simulink model "ASM_Traffic_A11"  (R2026a)
settings: Solver=ode1  StartTime=SIM.tstart.v  StopTime=SIM.tend.v  FixedStep=SIM.StepSize.v
PostLoadFcn:
  | if any(exist('dsrtsu_mdlpostloadfcn', 'file') ~= 0), dsrtsu_mdlpostloadfcn('Execute', bdroot); end
  | try, asm_mdl_postloadfcn(bdroot, 'UpdateModel', 3600); catch, disp(lasterr); end,
InitFcn:
  | , if any(exist('rtifpga_mdlclblib', 'file') ~= 0), rtifpga_mdlclblib('Init', bdroot); end,
  | , if any(exist('dsmpb_private', 'file') ~= 0), dsmpb_private('dsmpb_mdlclblib', 'Init', bdroot); end,
undefined symbols (not defined in the file): _to_, a0b2, ASM_BrakeHydraulics_DemoSystems, ASM_VehicleDynamics_DemoSystems, b98103fe8ad365046cd0, BrakeCircuit, controllerConfig, CPT, Crankshaft, DiscIntNeverNeededParam, dsmsi, FinalDriveAssembly, instance, MDL, ModeSignals, mu, Pos_BrakePedal_Maneuver, rad, RefSignals, s_to_rpm, SIM, SoftECU, Suspension, Tire, Transmission
libraries: ASM_Traffic_lib x135, simulink x98, ASM_Utils_lib x77, ASM_VehicleDynamics_lib x70, ASM_Environment_lib x22, dsmpblib x20, dsmsilib x15, MDLD_Utils_lib x10, ASM_BrakeHydraulics_lib x3, sl_discontinuities x2
(part 43 of 63)

== system ASM_Traffic_A11/VehicleDynamics/Plant/UserInterface/DISP_Plant/Velocities ==
  Velocities : Inport
  Angle_SideSlip_Vehicle[deg] : Subsystem
      mask Display: disp('')
  AngularVelocities : Scope  NumInputPorts=3
      settings: TimeSpan=5  ActiveDisplayYMinimum=43.2  ActiveDisplayYMaximum=45.1  DataLoggingMaxPoints=20000  DataLoggingDecimation=10  DataLoggingVariableName=ScopeData67
  Bus Selector2 : BusSelector  OutputSignals=Vehicle.Linear.v_Vehicle_CoG[x;y;z][km|h].v_x_Vehicle_CoG[km|h],Vehicle.Linear.v_Vehicle_CoG[x;y;z][km|h].v_y_Vehicle_CoG[km|h],Vehicle.Linear.v_Vehicle_CoG[x;y;z][km|h].v_z_Vehicle_CoG[km|h],Vehicle.Linear.Angle_SideSlip_Vehicle[deg],Vehicle.Angular.w_Vehicle_CoG[x;y;z][deg|s].RollRate_Vehicle_CoG[deg|s],Vehicle.Angular.w_Vehicle_CoG[x;y;z][deg|s].PitchRate_Vehicle_CoG[deg|s],Vehicle.Angular.w_Vehicle_CoG[x;y;z][deg|s].YawRate_Vehicle_CoG[deg|s]
  PitchRate_Vehicle_CoG[deg|s] : Subsystem
      mask Display: disp('')
  RollRate_Vehicle_CoG[deg|s] : Subsystem
      mask Display: disp('')
  TransVelocities : Scope  NumInputPorts=4
      settings: TimeSpan=5  ActiveDisplayYMinimum=-7.51344  ActiveDisplayYMaximum=67.07764  DataLoggingMaxPoints=20000  DataLoggingDecimation=10
  YawRate_Vehicle_CoG[deg|s] : Subsystem
      mask Display: disp('')
  v_x_Vehicle_CoG[km|h] : Subsystem
      mask Display: disp('')
  v_y_Vehicle_CoG[km|h] : Subsystem
      mask Display: disp('')
  v_z_Vehicle_CoG[km|h] : Subsystem
      mask Display: disp('')
  wires:
  Velocities/1 -> Bus Selector2/1
  RollRate_Vehicle_CoG[deg|s]/1(Out1) -> AngularVelocities/1  "RollRate_Vehicle_CoG[deg|s]"
  PitchRate_Vehicle_CoG[deg|s]/1(Out1) -> AngularVelocities/2  "PitchRate_Vehicle_CoG[deg|s]"
  YawRate_Vehicle_CoG[deg|s]/1(Out1) -> AngularVelocities/3  "YawRate_Vehicle_CoG[deg|s]"
  v_x_Vehicle_CoG[km|h]/1(Out1) -> TransVelocities/1  "v_x_Vehicle_CoG[km|h]"
  v_y_Vehicle_CoG[km|h]/1(Out1) -> TransVelocities/2  "v_y_Vehicle_CoG[km|h]"
  v_z_Vehicle_CoG[km|h]/1(Out1) -> TransVelocities/3  "v_z_Vehicle_CoG[km|h]"
  Angle_SideSlip_Vehicle[deg]/1(Out1) -> TransVelocities/4  "Angle_SideSlip_Vehicle[deg]"
  Bus Selector2/1 -> v_x_Vehicle_CoG[km|h]/1(In1)  "<v_x_Vehicle_CoG[km|h]>"
  Bus Selector2/2 -> v_y_Vehicle_CoG[km|h]/1(In1)  "<v_y_Vehicle_CoG[km|h]>"
  Bus Selector2/3 -> v_z_Vehicle_CoG[km|h]/1(In1)  "<v_z_Vehicle_CoG[km|h]>"
  Bus Selector2/4 -> Angle_SideSlip_Vehicle[deg]/1(In1)  "<Angle_SideSlip_Vehicle[deg]>"
  Bus Selector2/5 -> RollRate_Vehicle_CoG[deg|s]/1(In1)  "<RollRate_Vehicle_CoG[deg|s]>"
  Bus Selector2/6 -> PitchRate_Vehicle_CoG[deg|s]/1(In1)  "<PitchRate_Vehicle_CoG[deg|s]>"
  Bus Selector2/7 -> YawRate_Vehicle_CoG[deg|s]/1(In1)  "<YawRate_Vehicle_CoG[deg|s]>"

== system ASM_Traffic_A11/VehicleDynamics/Plant/UserInterface/DISP_Plant/WheelSpeeds ==
  WheelSpeeds : Inport
  Bus Selector2 : BusSelector  OutputSignals=WheelSpeed.omega_FL_Wheel[rad|s],WheelSpeed.omega_FR_Wheel[rad|s],WheelSpeed.omega_RL_Wheel[rad|s],WheelSpeed.omega_RR_Wheel[rad|s]
  WheelSpeeds1 : Scope  NumInputPorts=4
      settings: TimeSpan=5  ActiveDisplayYMinimum=8.14444E-18  ActiveDisplayYMaximum=9.00175E-18  DataLoggingMaxPoints=20000  DataLoggingDecimation=10
  omega_FL_Wheel[rad|s] : Subsystem
      mask Display: disp('')
  omega_FR_Wheel[rad|s] : Subsystem
      mask Display: disp('')
  omega_RL_Wheel[rad|s] : Subsystem
      mask Display: disp('')
  omega_RR_Wheel[rad|s] : Subsystem
      mask Display: disp('')
  wires:
  omega_RR_Wheel[rad|s]/1(Out1) -> WheelSpeeds1/4  "omega_RR_Wheel[rad|s]"
  omega_RL_Wheel[rad|s]/1(Out1) -> WheelSpeeds1/3  "omega_RL_Wheel[rad|s]"
  omega_FR_Wheel[rad|s]/1(Out1) -> WheelSpeeds1/2  "omega_FR_Wheel[rad|s]"
  omega_FL_Wheel[rad|s]/1(Out1) -> WheelSpeeds1/1  "omega_FL_Wheel[rad|s]"
  WheelSpeeds/1 -> Bus Selector2/1
  Bus Selector2/1 -> omega_FL_Wheel[rad|s]/1(In1)  "<omega_FL_Wheel[rad|s]>"
  Bus Selector2/2 -> omega_FR_Wheel[rad|s]/1(In1)  "<omega_FR_Wheel[rad|s]>"
  Bus Selector2/3 -> omega_RL_Wheel[rad|s]/1(In1)  "<omega_RL_Wheel[rad|s]>"
  Bus Selector2/4 -> omega_RR_Wheel[rad|s]/1(In1)  "<omega_RR_Wheel[rad|s]>"

== system ASM_Traffic_A11/VehicleDynamics/Plant/UserInterface/PAR_Plant/BrakeHydraulics_DistributionPattern_Switch ==
  Sw_DistributionPattern[1X|2II] : Constant
  Sw_DistributionPattern_[1X|2II] : Outport  VectorParamsAs1DForOutWhenUnconnected=off
  wires:
  Sw_DistributionPattern[1X|2II]/1 -> Sw_DistributionPattern_[1X|2II]/1  "Sw_DistributionPattern_[1X|2II]"

== system ASM_Traffic_A11/VehicleDynamics/Plant/UserInterface/PAR_Plant/Suspension_Inits ==
  Bus Creator1 : BusCreator  Inputs=2
  Mux : Mux
  Mux2 : Mux
  z_FL_Init[m] : Constant  Value=0  VectorParams1D=off
  z_FL_Init_dt[m|s] : Constant  Value=0  VectorParams1D=off
  z_FR_Init[m] : Constant  Value=0  VectorParams1D=off
  z_FR_Init_dt[m|s] : Constant  Value=0  VectorParams1D=off
  z_RL_Init[m] : Constant  Value=0  VectorParams1D=off
  z_RL_Init_dt[m|s] : Constant  Value=0  VectorParams1D=off
  z_RR_Init[m] : Constant  Value=0  VectorParams1D=off
  z_RR_Init_dt[m|s] : Constant  Value=0  VectorParams1D=off
  Suspension_Init : Outport  VectorParamsAs1DForOutWhenUnconnected=off
  wires:
  Mux2/1 -> Bus Creator1/1  "q_dt_Wheel_Init[:]"
  Mux/1 -> Bus Creator1/2  "q_Wheel_Init[:]"
  Bus Creator1/1 -> Suspension_Init/1  "Suspension_Init"
  z_FL_Init_dt[m|s]/1 -> Mux2/1
  z_FR_Init_dt[m|s]/1 -> Mux2/2
  z_RL_Init_dt[m|s]/1 -> Mux2/3
  z_RR_Init_dt[m|s]/1 -> Mux2/4
  z_FL_Init[m]/1 -> Mux/1
  z_FR_Init[m]/1 -> Mux/2
  z_RL_Init[m]/1 -> Mux/3
  z_RR_Init[m]/1 -> Mux/4

== system ASM_Traffic_A11/VehicleDynamics/Plant/UserInterface/PAR_Plant/Tire_Switches ==
  Bus Creator1 : BusCreator  Inputs=2
  Sw_r_Tire[1:intern;2:extern] : Constant  VectorParams1D=off
  r_Tire_extern[m] : Constant  Value=0.31  VectorParams1D=off
  Tire_Switches : Outport  VectorParamsAs1DForOutWhenUnconnected=off
  wires:
  Bus Creator1/1 -> Tire_Switches/1
  Sw_r_Tire[1:intern;2:extern]/1 -> Bus Creator1/1  "Sw_r_Tire[1:intern;2:extern]"
  r_Tire_extern[m]/1 -> Bus Creator1/2  "r_Tire_extern[m]"

== system ASM_Traffic_A11/VehicleDynamics/Plant/VehicleDynamics/ASMSignalCollector/Driving_Resistances ==
  F_Vehicle_Gravitational[x;y;z][N] : Inport
  Coef_RollingRes_Mean[] : Inport  Port=2
  F_x_Aero_CoorSys_V[N] : Inport  Port=3
  Bus Creator : BusCreator  Inputs=1
  Gain : Gain  Gain=-1
  Gain1 : Gain
  Gain2 : Gain
  Product : Product
  Sum : Sum  Inputs=+++
  X_Component : Selector  InputPortWidth=3  IndexOptions=Index vector (dialog)  Indices=[1]  OutputSizes=1
  Z_Component : Selector  InputPortWidth=3  IndexOptions=Index vector (dialog)  Indices=[3]  OutputSizes=1
  F_Driving_Res[N] : Outport  VectorParamsAs1DForOutWhenUnconnected=off
  wires:
  Gain/1 -> Bus Creator/1  "F_Driving_Res[N]"
  Sum/1 -> Gain/1
  Gain1/1 -> Sum/2  "F_Slope[N]"
  Gain2/1 -> Sum/1  "F_Aerodynamics[N]"
  Product/1 -> Sum/3  "F_Roll[N]"
  X_Component/1 -> Gain1/1
  Z_Component/1 -> Product/1
  Coef_RollingRes_Mean[]/1 -> Product/2
  F_x_Aero_CoorSys_V[N]/1 -> Gain2/1
  F_Vehicle_Gravitational[x;y;z][N]/1 -> Z_Component/1, X_Component/1
  Bus Creator/1 -> F_Driving_Res[N]/1  "DrivingResistances"

== system ASM_Traffic_A11/VehicleDynamics/Plant/VehicleDynamics/Brake/ASMSignalCollector ==
  BusCreator3 : BusCreator  Inputs=5
  ASMSignalBus : Outport  VectorParamsAs1DForOutWhenUnconnected=off
  wires:
  [ASMBUS_VehicleDynamics_Manifold] -> BusCreator3/5
  [ASMBUS_VehicleDynamics_VacuumServo] -> BusCreator3/4
  [ASMBUS_VehicleDynamics_BrakeDisc] -> BusCreator3/3
  [TAG_DISP_BrkHyd_MasterBrakeCylinder] -> BusCreator3/1
  [ASMBUS_VehicleDynamics_BrakeHydraulics] -> BusCreator3/2
  BusCreator3/1 -> ASMSignalBus/1  "Brake"

== system ASM_Traffic_A11/VehicleDynamics/Plant/VehicleDynamics/Brake/BRAKE_HYDRAULICS ==
  p_MasterBrakeCylinder[bar] : Inport
  Sw_DistributionPattern[1X|2II] : Inport  Port=2
  Reset[] : Inport  Port=3
  Ctrl_HydPump[0_1] : Inport  Port=4
  Ctrl_PreChargeValve_1[] : Inport  Port=5
  Ctrl_PreChargeValve_2[] : Inport  Port=6
  Ctrl_ChangeOverValve_1[] : Inport  Port=7
  Ctrl_ChangeOverValve_2[] : Inport  Port=8
  Ctrl_InletValve_FL[] : Inport  Port=9
  Ctrl_InletValve_FR[] : Inport  Port=10
  Ctrl_InletValve_RL[] : Inport  Port=11
  Ctrl_InletValve_RR[] : Inport  Port=12
  Ctrl_OutletValve_FL[] : Inport  Port=13
  Ctrl_OutletValve_FR[] : Inport  Port=14
  Ctrl_OutletValve_RL[] : Inport  Port=15
  Ctrl_OutletValve_RR[] : Inport  Port=16
  ECU_Mode[0None|1ABS|2ESP|3ASR] : Inport  Port=17
  p_Ambient[bar] : Inport  Port=18
  ASMSignalCollector : Subsystem
  BRAKING_CIRCUIT_BASIC : ASM_BrakeHydraulics_lib/BrakeHydraulics/BrakingCircuitBasic/BRAKING_CIRCUIT_BASIC  Tag=ASM_SUBCOMPONENT  Const_TimeConst=MDL.BrkHyd.BrakeHydraulicsBasic.Const_TimeConst  StepSize=SIM.StepSize  ASMProperties=struct('Name','BRAKING_CIRCUIT_BASIC','Version','4.0','Library','ASM_BrakeHydraulics_lib')  ASMInstanceName=braking_circuit_basic  ASMInstanceID=1
  Mux : Mux
  Mux1 : Mux
  Terminator_{1..2,4,8,11,14} (6 alike) : Terminator
  ASMSignalBus : Outport  VectorParamsAs1DForOutWhenUnconnected=off
  p_Brake[FL,FR,RL,RR][bar] : Outport  Port=2  VectorParamsAs1DForOutWhenUnconnected=off
  tag scope: TAG_DISP_BrkHyd_BrakingCircuitBasic=global
  wires:
  p_MasterBrakeCylinder[bar]/1 -> BRAKING_CIRCUIT_BASIC/1
  p_Ambient[bar]/1 -> BRAKING_CIRCUIT_BASIC/3
  Mux1/1 -> BRAKING_CIRCUIT_BASIC/6
  Mux/1 -> BRAKING_CIRCUIT_BASIC/5
  Ctrl_OutletValve_FL[]/1 -> Mux1/1
  Ctrl_OutletValve_FR[]/1 -> Mux1/2
  Ctrl_OutletValve_RL[]/1 -> Mux1/3
  Ctrl_OutletValve_RR[]/1 -> Mux1/4
  Ctrl_InletValve_RR[]/1 -> Mux/4
  Ctrl_InletValve_RL[]/1 -> Mux/3
  Ctrl_InletValve_FR[]/1 -> Mux/2
  Ctrl_InletValve_FL[]/1 -> Mux/1
  ECU_Mode[0None|1ABS|2ESP|3ASR]/1 -> BRAKING_CIRCUIT_BASIC/4
  Ctrl_ChangeOverValve_2[]/1 -> Terminator_8/1
  Ctrl_PreChargeValve_2[]/1 -> Terminator_11/1
  Ctrl_ChangeOverValve_1[]/1 -> Terminator_2/1
  Ctrl_PreChargeValve_1[]/1 -> Terminator_1/1
  Ctrl_HydPump[0_1]/1 -> Terminator_4/1
  ASMSignalCollector/1(ASMSignalBus) -> ASMSignalBus/1
  Reset[]/1 -> BRAKING_CIRCUIT_BASIC/2
  BRAKING_CIRCUIT_BASIC/1 -> [TAG_DISP_BrkHyd_BrakingCircuitBasic]
  BRAKING_CIRCUIT_BASIC/2 -> p_Brake[FL,FR,RL,RR][bar]/1
  Sw_DistributionPattern[1X|2II]/1 -> Terminator_14/1

== system ASM_Traffic_A11/VehicleDynamics/Plant/VehicleDynamics/Brake/ForceParkingBrake ==
  Sw_ParkingBrake[0Off|1On] : Inport
  F_ParkingBrake_Off[FL;FR;RL;RR][N] : Constant  Value=[0, 0, 0, 0]
  F_ParkingBrake_On[FL;FR;RL;RR][N] : Constant  Value=[0, 0, 10000, 10000]
  Switch : Switch  Threshold=0.5  SaturateOnIntegerOverflow=off  InputSameDT=off
  F_ParkingBrake[FL;FR;RL;RR][N] : Outport  VectorParamsAs1DForOutWhenUnconnected=off
  wires:
  Sw_ParkingBrake[0Off|1On]/1 -> Switch/2
  F_ParkingBrake_Off[FL;FR;RL;RR][N]/1 -> Switch/3
  F_ParkingBrake_On[FL;FR;RL;RR][N]/1 -> Switch/1
  Switch/1 -> F_ParkingBrake[FL;FR;RL;RR][N]/1

== system ASM_Traffic_A11/VehicleDynamics/Plant/VehicleDynamics/Brake/avoid_incomplete_trace2source ==
  In1 : Inport
  DummyGain : Gain
  Out1 : Outport
  wires:
  DummyGain/1 -> Out1/1
  In1/1 -> DummyGain/1

== system ASM_Traffic_A11/VehicleDynamics/Plant/VehicleDynamics/Brake/avoid_incomplete_trace2source1 ==
  In1 : Inport
  DummyGain : Gain
  Out1 : Outport
  wires:
  In1/1 -> DummyGain/1
  DummyGain/1 -> Out1/1

== system ASM_Traffic_A11/VehicleDynamics/Plant/VehicleDynamics/Brake/avoid_incomplete_trace2source2 ==
  In1 : Inport
  DummyGain : Gain
  Out1 : Outport
  wires:
  DummyGain/1 -> Out1/1
  In1/1 -> DummyGain/1

== system ASM_Traffic_A11/VehicleDynamics/Plant/VehicleDynamics/CommonVehicleParameters/Rename1 ==
  In1 : Inport
  Out1 : Outport  VectorParamsAs1DForOutWhenUnconnected=off
  wires:
  In1/1 -> Out1/1

== system ASM_Traffic_A11/VehicleDynamics/Plant/VehicleDynamics/CommonVehicleParameters/Rename2 ==
  In1 : Inport
  Out1 : Outport  VectorParamsAs1DForOutWhenUnconnected=off
  wires:
  In1/1 -> Out1/1

== system ASM_Traffic_A11/VehicleDynamics/Plant/VehicleDynamics/CommonVehicleParameters/Rename3 ==
  In1 : Inport
  Out1 : Outport  VectorParamsAs1DForOutWhenUnconnected=off
  wires:
  In1/1 -> Out1/1

== system ASM_Traffic_A11/VehicleDynamics/Plant/VehicleDynamics/CommonVehicleParameters/Rename4 ==
  In1 : Inport
  Out1 : Outport  VectorParamsAs1DForOutWhenUnconnected=off
  wires:
  In1/1 -> Out1/1

== system ASM_Traffic_A11/VehicleDynamics/Plant/VehicleDynamics/CommonVehicleParameters/Rename5 ==
  In1 : Inport
  Out1 : Outport  VectorParamsAs1DForOutWhenUnconnected=off
  wires:
  In1/1 -> Out1/1

== system ASM_Traffic_A11/VehicleDynamics/Plant/VehicleDynamics/CommonVehicleParameters/Rename6 ==
  In1 : Inport
  Out1 : Outport  VectorParamsAs1DForOutWhenUnconnected=off
  wires:
  In1/1 -> Out1/1

== system ASM_Traffic_A11/VehicleDynamics/Plant/VehicleDynamics/CommonVehicleParameters/Rename7 ==
  In1 : Inport
  Out1 : Outport  VectorParamsAs1DForOutWhenUnconnected=off
  wires:
  In1/1 -> Out1/1

== system ASM_Traffic_A11/VehicleDynamics/Plant/VehicleDynamics/CommonVehicleParameters/Rename8 ==
  In1 : Inport
  Out1 : Outport  VectorParamsAs1DForOutWhenUnconnected=off
  wires:
  In1/1 -> Out1/1

== system ASM_Traffic_A11/VehicleDynamics/Plant/VehicleDynamics/Exchangeable_Plant_Signals/ASMInterface_RollerDyno ==
  Angle_Gamma_FL_Wheel[deg] : Inport
  omega_Wheel[rad|s] : Inport  Port=2
  Bus Creator6 : BusCreator  Inputs=2
  Out : Outport  VectorParamsAs1DForOutWhenUnconnected=off
  wires:
  Bus Creator6/1 -> Out/1  "RollerDyno"
  omega_Wheel[rad|s]/1 -> Bus Creator6/2  "omega_Wheel[rad|s]"
  Angle_Gamma_FL_Wheel[deg]/1 -> Bus Creator6/1  "Angle_Gamma_FL_Wheel[deg]"

== system ASM_Traffic_A11/VehicleDynamics/Plant/VehicleDynamics/Exchangeable_Plant_Signals/ASMInterface_Steering ==
  Displ_Steering[m] : Inport
  Displ_Steering_dt[m|s] : Inport  Port=2
  Bus Creator6 : BusCreator  Inputs=2
  Out : Outport  VectorParamsAs1DForOutWhenUnconnected=off
  wires:
  Displ_Steering_dt[m|s]/1 -> Bus Creator6/2  "Displ_Steering_dt[m|s]"
  Displ_Steering[m]/1 -> Bus Creator6/1  "Displ_Steering[m]"
  Bus Creator6/1 -> Out/1  "Steering"

== system ASM_Traffic_A11/VehicleDynamics/Plant/VehicleDynamics/Suspension/ASMSignalCollector ==
  BusCreator1 : BusCreator  Inputs=2
  ASMSignalBus : Outport  VectorParamsAs1DForOutWhenUnconnected=off
  wires:
  BusCreator1/1 -> ASMSignalBus/1  "Suspension"
  [ASMBUS_SuspensionFront] -> BusCreator1/1
  [ASMBUS_SuspensionRear] -> BusCreator1/2

== system ASM_Traffic_A11/VehicleDynamics/Plant/VehicleDynamics/Suspension/SuspensionFront ==
  q_Wheel_dt[q1_Front;q2_Front;q1_Rear;q2_Rear][] : Inport
  q_Wheel[q1_Front;q2_Front;q1_Rear;q2_Rear][] : Inport  Port=2
  F_Tire[FL;FR;RL;RR][x;y;z][N] : Inport  Port=3
  Trq_Tire[FL;FR;RL;RR][x;y;z][Nm] : Inport  Port=4
  AirSuspensionSignals_In : Inport  Port=5
  Reset[] : Inport  Port=6
  Sw_Rotation[1Cardan|2ToeCamberCaster] : Inport  Port=7
  Displ_SteeringRod_dt[m|s] : Inport  Port=8  PortDimensions=1
  Displ_SteeringRod[m] : Inport  Port=9  PortDimensions=1
  ASMSignalCollector : Subsystem
  Bus Creator1 : BusCreator  Inputs=8
  Bus Creator : BusCreator  Inputs=3
  Constant : Constant  Value=0
  Constant1 : Constant  Value=[0;0]
  Constant2 : Constant  Value=0
  Constant3 : Constant  Value=[0;0;0]
  Demux : Demux  Outputs=[1 1]
      settings: DisplayOption=none
  F_FL_dDispl_external[N|m] : Constant  Value=0
  F_FL_external[N] : Constant  Value=0
  F_FR_dDispl_external[N|m] : Constant  Value=0
  F_FR_external[N] : Constant  Value=0
  Goto Tag Visibility : GotoTagVisibility  GotoTag=ASMBUS_SuspensionComplianceFront
  Goto Tag Visibility1 : GotoTagVisibility  GotoTag=ASMBUS_SuspensionKinematicsFront
  Goto Tag Visibility2 : GotoTagVisibility  GotoTag=ASMBUS_WheelRelativeVelocityFront
  Goto Tag Visibility3 : GotoTagVisibility  GotoTag=ASMBUS_WheelRelativePositionFront
  Goto Tag Visibility4 : GotoTagVisibility  GotoTag=ASMBUS_SuspensionForcesFront
  Goto Tag Visibility5 : GotoTagVisibility  GotoTag=ASMBUS_SuspensionForcesKinematicsFront
  Mux : Mux  Inputs=2
  Mux1 : Mux  Inputs=2
  Mux2 : Mux  Inputs=2
  OpenSusKin : ASM_Utils_lib/Miscellaneous/OpenSystem  popupLibBlk=<select here>  popupTargetDemo=<select here>  Demosystem=VehicleDynamics_Suspension  variantLib=ASM_VehicleDynamics_DemoSystems/Suspension
  RELATIVE_POSITION_FRONT : ASM_VehicleDynamics_lib/VehicleDynamics/Suspension/Front/CommonSuspensionBlocks/RELATIVE_POSITION_FRONT  Tag=ASM_SUBCOMPONENT  ASMProperties=struct('Name','RELATIVE_POSITION_FRONT','Version','6.0','Library','ASM_VehicleDynamics_lib')  ASMInstanceName=relative_position_front  ASMInstanceID=1
  RELATIVE_VELOCITIES_FRONT : ASM_VehicleDynamics_lib/VehicleDynamics/Suspension/Front/CommonSuspensionBlocks/RELATIVE_VELOCITIES_FRONT  Tag=ASM_SUBCOMPONENT  ASMProperties=struct('Name','RELATIVE_VELOCITIES_FRONT','Version','4.0','Library','ASM_VehicleDynamics_lib')  ASMInstanceName=relative_velocities_front  ASMInstanceID=1
  STABI_COMP_FRONT : ASM_VehicleDynamics_lib/VehicleDynamics/Suspension/Front/CommonSuspensionBlocks/STABI_COMP_FRONT  ASMProperties=struct('Name','STABI_COMP_FRONT','Version','1.0','Library','ASM_VehicleDynamics_lib')  ASMInstanceName=stabi_comp_front  ASMInstanceID=1
  SUSCOMP_2D_FRONT : ASM_VehicleDynamics_lib/VehicleDynamics/Suspension/Front/CommonSuspensionBlocks/SUSCOMP_2D_FRONT  Tag=ASM_SUBCOMPONENT  Map_Displ_x_Wheel_F_x=MDL.VehicleDynamics.SuspensionCompliance.Front.Map_Displ_x_Wheel_F_x_2d  Map_Displ_x_Wheel_F_y=MDL.VehicleDynamics.SuspensionCompliance.Front.Map_Displ_x_Wheel_F_y_2d  Map_Displ_x_Wheel_Trq_x=MDL.VehicleDynamics.SuspensionCompliance.Front.Map_Displ_x_Wheel_Trq_x_2d  Map_Displ_x_Wheel_Trq_y=MDL.VehicleDynamics.SuspensionCompliance.Front.Map_Displ_x_Wheel_Trq_y_2d  Map_Displ_x_Wheel_Trq_z=MDL.VehicleDynamics.SuspensionCompliance.Front.Map_Displ_x_Wheel_Trq_z_2d  Map_Displ_y_Wheel_F_x=MDL.VehicleDynamics.SuspensionCompliance.Front.Map_Displ_y_Wheel_F_x_2d  Map_Displ_y_Wheel_F_y=MDL.VehicleDynamics.SuspensionCompliance.Front.Map_Displ_y_Wheel_F_y_2d  Map_Displ_y_Wheel_Trq_x=MDL.VehicleDynamics.SuspensionCompliance.Front.Map_Displ_y_Wheel_Trq_x_2d  Map_Displ_y_Wheel_Trq_y=MDL.VehicleDynamics.SuspensionCompliance.Front.Map_Displ_y_Wheel_Trq_y_2d  Map_Displ_y_Wheel_Trq_z=MDL.VehicleDynamics.SuspensionCompliance.Front.Map_Displ_y_Wheel_Trq_z_2d  Map_Angle_Alpha_Wheel_F_x=MDL.VehicleDynamics.SuspensionCompliance.Front.Map_Angle_AlphaCamber_Wheel_F_x_2d  Map_Angle_Alpha_Wheel_F_y=MDL.VehicleDynamics.SuspensionCompliance.Front.Map_Angle_AlphaCamber_Wheel_F_y_2d  Map_Angle_Alpha_Wheel_Trq_x=MDL.VehicleDynamics.SuspensionCompliance.Front.Map_Angle_AlphaCamber_Wheel_Trq_x_2d  Map_Angle_Alpha_Wheel_Trq_y=MDL.VehicleDynamics.SuspensionCompliance.Front.Map_Angle_AlphaCamber_Wheel_Trq_y_2d  Map_Angle_Alpha_Wheel_Trq_z=MDL.VehicleDynamics.SuspensionCompliance.Front.Map_Angle_AlphaCamber_Wheel_Trq_z_2d  Map_Angle_Gamma_Wheel_F_x=MDL.VehicleDynamics.SuspensionCompliance.Front.Map_Angle_GammaToe_Wheel_F_x_2d  Map_Angle_Gamma_Wheel_F_y=MDL.VehicleDynamics.SuspensionCompliance.Front.Map_Angle_GammaToe_Wheel_F_y_2d  Map_Angle_Gamma_Wheel_Trq_x=MDL.VehicleDynamics.SuspensionCompliance.Front.Map_Angle_GammaToe_Wheel_Trq_x_2d  Map_Angle_Gamma_Wheel_Trq_y=MDL.VehicleDynamics.SuspensionCompliance.Front.Map_Angle_GammaToe_Wheel_Trq_y_2d  Map_Angle_Gamma_Wheel_Trq_z=MDL.VehicleDynamics.SuspensionCompliance.Front.Map_Angle_GammaToe_Wheel_Trq_z_2d  Const_NaturalFrequency_Displ_x=MDL.VehicleDynamics.SuspensionCompliance.Front.Const_NaturalFrequency_Displ_x  Const_NaturalFrequency_Displ_y=MDL.VehicleDynamics.SuspensionCompliance.Front.Const_NaturalFrequency_Displ_y  Const_NaturalFrequency_Angle_Alpha=MDL.VehicleDynamics.SuspensionCompliance.Front.Const_NaturalFrequency_Angle_AlphaCamber  Const_NaturalFrequency_Angle_Gamma=MDL.VehicleDynamics.SuspensionCompliance.Front.Const_NaturalFrequency_Angle_GammaToe  StepSize=SIM.StepSize  ASMProperties=struct('Name','SUSCOMP_2D_FRONT','Version','4.0','Library','ASM_VehicleDynamics_lib')  ASMInstanceName=suscomp_2d_front  ASMInstanceID=1
  SUSPENSION_FORCES_FRONT : ASM_VehicleDynamics_lib/VehicleDynamics/Suspension/Front/CommonSuspensionBlocks/SUSPENSION_FORCES_FRONT  Tag=ASM_SUBCOMPONENT  Map_Force_Left_Spring=MDL.VehicleDynamics.Suspension.Front.Map_Force_LeftSpring  Map_Force_Left_Damper=MDL.VehicleDynamics.Suspension.Front.Map_Force_LeftDamper  Map_Force_Right_Spring=MDL.VehicleDynamics.Suspension.Front.Map_Force_RightSpring  Map_Force_Right_Damper=MDL.VehicleDynamics.Suspension.Front.Map_Force_RightDamper  Map_Force_Stabilizer=MDL.VehicleDynamics.Suspension.Front.Map_Force_Stabilizer  ASMProperties=struct('Name','SUSPENSION_FORCES_FRONT','Version','4.0','Library','ASM_VehicleDynamics_lib')  ASMInstanceName=SusForcesFront  ASMInstanceID=1
  SUSPENSION_FORCE_KINEMATICS_FRONT : ASM_VehicleDynamics_lib/VehicleDynamics/Suspension/Front/CommonSuspensionBlocks/SUSPENSION_FORCE_KINEMATICS_FRONT  Tag=ASM_SUBCOMPONENT  StepSize=SIM.StepSize  ASMProperties=struct('Name','SUSPENSION_FORCE_KINEMATICS_FRONT','Version','5.0','Library','ASM_VehicleDynamics_lib')  ASMInstanceName=suspension_force_kinematics_front  ASMInstanceID=1
  Selector : Selector  InputPortWidth=4  IndexOptions=Index vector (dialog)  Indices=[1 2]  OutputSizes=1
  Selector1 : Selector  InputPortWidth=12  IndexOptions=Index vector (dialog)  Indices=[1 4]  OutputSizes=1
  Selector10 : Selector  InputPortWidth=12  IndexOptions=Index vector (dialog)  Indices=[1 4]  OutputSizes=1
  Selector2 : Selector  InputPortWidth=12  IndexOptions=Index vector (dialog)  Indices=[2 5]  OutputSizes=1
  Selector3 : Selector  InputPortWidth=12  IndexOptions=Index vector (dialog)  Indices=[3 6]  OutputSizes=1
  Selector4 : Selector  InputPortWidth=12  IndexOptions=Index vector (dialog)  Indices=[2 5]  OutputSizes=1
  Selector8 : Selector  InputPortWidth=4  IndexOptions=Index vector (dialog)  Indices=[1 2]  OutputSizes=1
  Sum{,1..3} (4 alike) : Sum  Inputs=++|
  Sum4 : Sum  Inputs=|++
  SusKin_Front : Subsystem  Tag=VehicleDynamics_Suspension
  Terminator : Terminator
  zeros : Constant  Value=zeros(6,1)
  "Pos_Wheel[FL,FR][x;y;z][m] " : Outport  VectorParamsAs1DForOutWhenUnconnected=off
  UnitVec_y_Wheel_CoorSys_V[FL,FR][x;y;z] : Outport  Port=2  VectorParamsAs1DForOutWhenUnconnected=off
  v_Rel_WheelBody[FL,FR][x;y;z][m|s] : Outport  Port=3  VectorParamsAs1DForOutWhenUnconnected=off
  w_Rel_WheelBody[FL,FR][x;y;z][rad|s] : Outport  Port=4  VectorParamsAs1DForOutWhenUnconnected=off
  gF_Front_Susp[q1,q2][] : Outport  Port=5  VectorParamsAs1DForOutWhenUnconnected=off
  gFront_dq_Front_dt[2x2][] : Outport  Port=6  VectorParamsAs1DForOutWhenUnconnected=off
  SuspensionKinematicRelations_Front : Outport  Port=7  VectorParamsAs1DForOutWhenUnconnected=off
  AirSuspensionSignals_Front : Outport  Port=8  VectorParamsAs1DForOutWhenUnconnected=off
  ASMSignalBus : Outport  Port=9  VectorParamsAs1DForOutWhenUnconnected=off
  tag scope: ASMBUS_SuspensionComplianceFront=scoped, ASMBUS_SuspensionForcesFront=scoped, ASMBUS_SuspensionForcesKinematicsFront=scoped, ASMBUS_SuspensionKinematicsFront=scoped, ASMBUS_WheelRelativePositionFront=scoped, ASMBUS_WheelRelativeVelocityFront=scoped
  wires:
  SusKin_Front/24(Displ_Stabilizer_dSteering[Left;Right][]) -> Bus Creator/3  "Displ_Stabi_dSteering[Left;Right]"
  Bus Creator/1 -> STABI_COMP_FRONT/1  "Displ_dSteering[Spring;Damper;Stabi]"
  SusKin_Front/23(Displ_Damper_dSteering[Left;Right][]) -> Bus Creator/2  "Displ_Damper_dSteering[Left;Right]"
  SusKin_Front/22(Displ_Spring_dSteering[Left;Right][]) -> Bus Creator/1  "Displ_Spring_dSteering[Left;Right]"
  Constant3/1 -> SusKin_Front/5(WheelPos_Offset[x;y;z][m])
  SUSPENSION_FORCES_FRONT/1 -> [ASMBUS_SuspensionForcesFront]
  SUSCOMP_2D_FRONT/1 -> [ASMBUS_SuspensionComplianceFront]
  Mux2/1 -> SusKin_Front/2(Displ_SteeringRod_dt[Left;Right][m|s]), RELATIVE_VELOCITIES_FRONT/1
  F_Tire[FL;FR;RL;RR][x;y;z][N]/1 -> Selector1/1, Selector2/1
  RELATIVE_VELOCITIES_FRONT/1 -> [ASMBUS_WheelRelativeVelocityFront]
  SUSCOMP_2D_FRONT/2 -> RELATIVE_VELOCITIES_FRONT/4
  SUSCOMP_2D_FRONT/3 -> RELATIVE_VELOCITIES_FRONT/5
  SUSCOMP_2D_FRONT/4 -> RELATIVE_VELOCITIES_FRONT/6
  SUSCOMP_2D_FRONT/5 -> RELATIVE_VELOCITIES_FRONT/7
  SUSCOMP_2D_FRONT/6 -> RELATIVE_POSITION_FRONT/1
  SUSCOMP_2D_FRONT/7 -> RELATIVE_POSITION_FRONT/2
  SUSCOMP_2D_FRONT/8 -> RELATIVE_POSITION_FRONT/3
  SUSCOMP_2D_FRONT/9 -> RELATIVE_POSITION_FRONT/4
  SusKin_Front/10(Pos_Left_Wheel[x;y;z][m]) -> RELATIVE_POSITION_FRONT/5
  SusKin_Front/11(Pos_Right_Wheel[x;y;z][m]) -> RELATIVE_POSITION_FRONT/6
  SusKin_Front/12(UnitVec_y_Wheel_Left[x;y;z]) -> RELATIVE_POSITION_FRONT/7
  SusKin_Front/13(UnitVec_y_Wheel_Right[x;y;z]) -> RELATIVE_POSITION_FRONT/8
  SusKin_Front/14(Displ_Spring[Left;Right][m]) -> SUSPENSION_FORCES_FRONT/1
  SusKin_Front/15(Displ_Damper_dt[Left;Right][m|s]) -> SUSPENSION_FORCES_FRONT/2
  SusKin_Front/16(Displ_Stabilizer[m]) -> SUSPENSION_FORCES_FRONT/3
  SUSPENSION_FORCES_FRONT/2 -> Sum/2
  SUSPENSION_FORCES_FRONT/3 -> Sum1/2
  SUSPENSION_FORCES_FRONT/4 -> SUSPENSION_FORCE_KINEMATICS_FRONT/3
  SUSPENSION_FORCES_FRONT/5 -> SUSPENSION_FORCE_KINEMATICS_FRONT/4
  SUSPENSION_FORCES_FRONT/6 -> STABI_COMP_FRONT/4, SUSPENSION_FORCE_KINEMATICS_FRONT/5
  SUSPENSION_FORCES_FRONT/7 -> SUSPENSION_FORCE_KINEMATICS_FRONT/6
  SUSPENSION_FORCES_FRONT/8 -> Sum2/2
  SUSPENSION_FORCES_FRONT/9 -> Sum3/2
  SUSPENSION_FORCES_FRONT/10 -> SUSPENSION_FORCE_KINEMATICS_FRONT/9
  SUSPENSION_FORCES_FRONT/11 -> SUSPENSION_FORCE_KINEMATICS_FRONT/10
  SusKin_Front/17(Displ_Spring_Left_dq[qL;qR][]) -> SUSPENSION_FORCE_KINEMATICS_FRONT/11
  SusKin_Front/18(Displ_Damper_Left_dq[qL;qR][]) -> SUSPENSION_FORCE_KINEMATICS_FRONT/12
  SusKin_Front/19(Displ_Stabilizer_dq[qL;qR][]) -> SUSPENSION_FORCE_KINEMATICS_FRONT/13
  SusKin_Front/20(Displ_Spring_Right_dq[qL;qR][]) -> SUSPENSION_FORCE_KINEMATICS_FRONT/14
  SusKin_Front/21(Displ_Damper_Right_dq[qL;qR][]) -> SUSPENSION_FORCE_KINEMATICS_FRONT/15
  RELATIVE_POSITION_FRONT/2 -> "Pos_Wheel[FL,FR][x;y;z][m] "/1
  RELATIVE_POSITION_FRONT/3 -> UnitVec_y_Wheel_CoorSys_V[FL,FR][x;y;z]/1
  SUSPENSION_FORCE_KINEMATICS_FRONT/3 -> Mux1/2
  Mux1/1 -> gF_Front_Susp[q1,q2][]/1
  SUSPENSION_FORCE_KINEMATICS_FRONT/4 -> gFront_dq_Front_dt[2x2][]/1
  Mux/1 -> SusKin_Front/1(Displ_SteeringRod[Left;Right][m])
  q_Wheel_dt[q1_Front;q2_Front;q1_Rear;q2_Rear][]/1 -> Selector/1
  q_Wheel[q1_Front;q2_Front;q1_Rear;q2_Rear][]/1 -> Selector8/1
  SusKin_Front/2(Pos_Left_Wheel_dq[qL;qR][x;y;z][]) -> RELATIVE_VELOCITIES_FRONT/8, Bus Creator1/1  "Pos_FL_Wheel_dq_Front[q1;q2][x;y;z][]"
  SusKin_Front/3(Pos_Left_Wheel_dDispl_SteeringRod[x;y;z][]) -> RELATIVE_VELOCITIES_FRONT/9, Bus Creator1/2  "Pos_FL_Wheel_dDispl_SteeringRod[x;y;z][]"
  SusKin_Front/4(w_Rel_Left_Wheel_dq_dt[qL;qR][x;y;z][rad|m]) -> RELATIVE_VELOCITIES_FRONT/10, Bus Creator1/3  "w_Rel_FL_Wheel_dq_Front_dt[q1;q2][x;y;z][]"
  SusKin_Front/5(w_Rel_Left_Wheel_dDispl_SteeringRod_dt[x;y;z][rad|m]) -> RELATIVE_VELOCITIES_FRONT/11, STABI_COMP_FRONT/2, Bus Creator1/4  "w_Rel_FL_Wheel_dDispl_SteeringRod_dt[x;y;z][rad|m]"
  SusKin_Front/6(Pos_Right_Wheel_dq[qL;qR][x;y;z][]) -> RELATIVE_VELOCITIES_FRONT/12, Bus Creator1/5  "Pos_FR_Wheel_dq_Front[q1;q2][x;y;z][]"
  SusKin_Front/7(Pos_Right_Wheel_dDispl_SteeringRod[x;y;z][]) -> RELATIVE_VELOCITIES_FRONT/13, Bus Creator1/6  "Pos_FR_Wheel_dDispl_SteeringRod[x;y;z][]"
  SusKin_Front/8(w_Rel_Right_Wheel_dq_dt[qL;qR][x;y;z][rad|m]) -> RELATIVE_VELOCITIES_FRONT/14, Bus Creator1/7  "w_Rel_FR_Wheel_dq_Front[q1;q2][x;y;z][]"
  SusKin_Front/9(w_Rel_Right_Wheel_dDispl_SteeringRod_dt[x;y;z][rad|m]) -> RELATIVE_VELOCITIES_FRONT/15, STABI_COMP_FRONT/3, Bus Creator1/8  "w_Rel_FR_Wheel_dDispl_SteeringRod_dt[x;y;z][rad|m]"
  Bus Creator1/1 -> SuspensionKinematicRelations_Front/1  "SuspensionKinematicRelations_Front"
  RELATIVE_POSITION_FRONT/1 -> [ASMBUS_WheelRelativePositionFront]
  RELATIVE_VELOCITIES_FRONT/2 -> v_Rel_WheelBody[FL,FR][x;y;z][m|s]/1
  RELATIVE_VELOCITIES_FRONT/3 -> w_Rel_WheelBody[FL,FR][x;y;z][rad|s]/1
  Demux/2 -> RELATIVE_VELOCITIES_FRONT/3
  Demux/1 -> RELATIVE_VELOCITIES_FRONT/2
  SUSPENSION_FORCE_KINEMATICS_FRONT/1 -> [ASMBUS_SuspensionForcesKinematicsFront]
  SusKin_Front/1(ASMSignalBus) -> [ASMBUS_SuspensionKinematicsFront]
  SUSPENSION_FORCE_KINEMATICS_FRONT/2 -> Mux1/1
  Reset[]/1 -> SUSCOMP_2D_FRONT/6
  Constant/1 -> SUSPENSION_FORCE_KINEMATICS_FRONT/16, SUSPENSION_FORCE_KINEMATICS_FRONT/17, SUSPENSION_FORCE_KINEMATICS_FRONT/18, SUSPENSION_FORCE_KINEMATICS_FRONT/19
  Trq_Tire[FL;FR;RL;RR][x;y;z][Nm]/1 -> Selector10/1, Selector4/1, Selector3/1
  Constant1/1 -> SUSPENSION_FORCE_KINEMATICS_FRONT/20, SUSPENSION_FORCE_KINEMATICS_FRONT/21
  Displ_SteeringRod[m]/1 -> Mux/2, Mux/1
  Displ_SteeringRod_dt[m|s]/1 -> Mux2/2, Mux2/1
  Sw_Rotation[1Cardan|2ToeCamberCaster]/1 -> SusKin_Front/6(Sw_Rotation[1Cardan|2ToeCamberSideView]), SUSCOMP_2D_FRONT/7, RELATIVE_POSITION_FRONT/9
  zeros/1 -> SUSCOMP_2D_FRONT/8
  Selector/1 -> SusKin_Front/4(Displ_z_dt_Wheel[Left;Right][m|s]), Demux/1
  Selector8/1 -> SusKin_Front/3(Displ_z_Wheel[Left;Right][m])
  Selector1/1 -> SUSCOMP_2D_FRONT/1
  Selector2/1 -> SUSCOMP_2D_FRONT/2
  Selector10/1 -> SUSCOMP_2D_FRONT/3
  Sum/1 -> SUSPENSION_FORCE_KINEMATICS_FRONT/1
  F_FL_external[N]/1 -> Sum/1
  Sum1/1 -> SUSPENSION_FORCE_KINEMATICS_FRONT/2
  F_FL_dDispl_external[N|m]/1 -> Sum1/1
  F_FR_external[N]/1 -> Sum2/1
  F_FR_dDispl_external[N|m]/1 -> Sum3/1
  Sum2/1 -> SUSPENSION_FORCE_KINEMATICS_FRONT/7
  Sum3/1 -> SUSPENSION_FORCE_KINEMATICS_FRONT/8
  AirSuspensionSignals_In/1 -> Terminator/1
  Constant2/1 -> AirSuspensionSignals_Front/1
  Selector3/1 -> Sum4/1
  Sum4/1 -> SUSCOMP_2D_FRONT/5
  STABI_COMP_FRONT/1 -> Sum4/2
  Selector4/1 -> SUSCOMP_2D_FRONT/4
  ASMSignalCollector/1(SuspensionFront) -> ASMSignalBus/1

== system ASM_Traffic_A11/VehicleDynamics/Plant/VehicleDynamics/Suspension/SuspensionRear ==
  q_Wheel_dt[q1_Front;q2_Front;q1_Rear;q2_Rear][] : Inport
  q_Wheel[q1_Front;q2_Front;q1_Rear;q2_Rear][] : Inport  Port=2
  F_Tire[FL;FR;RL;RR][x;y;z][N] : Inport  Port=3
  Trq_Tire[FL;FR;RL;RR][x;y;z][Nm] : Inport  Port=4
  AirSuspensionSignals_In : Inport  Port=5
  Reset[] : Inport  Port=6
  Sw_Rotation[1Cardan|2ToeCamberCaster] : Inport  Port=7
  ASMSignalCollector : Subsystem
  Bus Creator : BusCreator  Inputs=8
  Constant : Constant  Value=[0 0]
  Constant1 : Constant  Value=0
  Constant2 : Constant  Value=0
  Constant3 : Constant  Value=[0;0]
  Demux : Demux  Outputs=[1 1]
      settings: DisplayOption=none
  F_RL_dDispl_external[N|m] : Constant  Value=0
  F_RL_external[N] : Constant  Value=0
  F_RR_dDispl_external[N|m] : Constant  Value=0
  F_RR_external[N] : Constant  Value=0
  Goto Tag Visibility : GotoTagVisibility  GotoTag=ASMBUS_SuspensionComplianceRear
  Goto Tag Visibility1 : GotoTagVisibility  GotoTag=ASMBUS_SuspensionKinematicsRear
  Goto Tag Visibility2 : GotoTagVisibility  GotoTag=ASMBUS_SuspensionRelativeVelocitiesRear
  Goto Tag Visibility3 : GotoTagVisibility  GotoTag=ASMBUS_SuspensionRelativePositionRear
  Goto Tag Visibility4 : GotoTagVisibility  GotoTag=ASMBUS_SuspensionForcesRear
  Goto Tag Visibility5 : GotoTagVisibility  GotoTag=ASMBUS_SuspensionForceKinematicsRear
  Mux1 : Mux  Inputs=2
  OpenSusKin : ASM_Utils_lib/Miscellaneous/OpenSystem  popupLibBlk=<select here>  popupTargetDemo=<select here>  Demosystem=VehicleDynamics_Suspension  variantLib=ASM_VehicleDynamics_DemoSystems/Suspension
  RELATIVE_POSITION_REAR : ASM_VehicleDynamics_lib/VehicleDynamics/Suspension/Rear/CommonSuspensionBlocks/RELATIVE_POSITION_REAR  Tag=ASM_SUBCOMPONENT  ASMProperties=struct('Name','RELATIVE_POSITION_REAR','Version','6.0','Library','ASM_VehicleDynamics_lib')  ASMInstanceName=relative_position_rear  ASMInstanceID=1
  RELATIVE_VELOCITIES_REAR : ASM_VehicleDynamics_lib/VehicleDynamics/Suspension/Rear/CommonSuspensionBlocks/RELATIVE_VELOCITIES_REAR  Tag=ASM_SUBCOMPONENT  ASMProperties=struct('Name','RELATIVE_VELOCITIES_REAR','Version','4.0','Library','ASM_VehicleDynamics_lib')  ASMInstanceName=relative_velocities_rear  ASMInstanceID=1
  SUSCOMP_2D_REAR : ASM_VehicleDynamics_lib/VehicleDynamics/Suspension/Rear/CommonSuspensionBlocks/SUSCOMP_2D_REAR  Tag=ASM_SUBCOMPONENT  Map_Displ_x_Wheel_F_x=MDL.VehicleDynamics.SuspensionCompliance.Rear.Map_Displ_x_Wheel_F_x_2d  Map_Displ_x_Wheel_F_y=MDL.VehicleDynamics.SuspensionCompliance.Rear.Map_Displ_x_Wheel_F_y_2d  Map_Displ_x_Wheel_Trq_x=MDL.VehicleDynamics.SuspensionCompliance.Rear.Map_Displ_x_Wheel_Trq_x_2d  Map_Displ_x_Wheel_Trq_y=MDL.VehicleDynamics.SuspensionCompliance.Rear.Map_Displ_x_Wheel_Trq_y_2d  Map_Displ_x_Wheel_Trq_z=MDL.VehicleDynamics.SuspensionCompliance.Rear.Map_Displ_x_Wheel_Trq_z_2d  Map_Displ_y_Wheel_F_x=MDL.VehicleDynamics.SuspensionCompliance.Rear.Map_Displ_y_Wheel_F_x_2d  Map_Displ_y_Wheel_F_y=MDL.VehicleDynamics.SuspensionCompliance.Rear.Map_Displ_y_Wheel_F_y_2d  Map_Displ_y_Wheel_Trq_x=MDL.VehicleDynamics.SuspensionCompliance.Rear.Map_Displ_y_Wheel_Trq_x_2d  Map_Displ_y_Wheel_Trq_y=MDL.VehicleDynamics.SuspensionCompliance.Rear.Map_Displ_y_Wheel_Trq_y_2d  Map_Displ_y_Wheel_Trq_z=MDL.VehicleDynamics.SuspensionCompliance.Rear.Map_Displ_y_Wheel_Trq_z_2d  Map_Angle_Alpha_Wheel_F_x=MDL.VehicleDynamics.SuspensionCompliance.Rear.Map_Angle_AlphaCamber_Wheel_F_x_2d  Map_Angle_Alpha_Wheel_F_y=MDL.VehicleDynamics.SuspensionCompliance.Rear.Map_Angle_AlphaCamber_Wheel_F_y_2d  Map_Angle_Alpha_Wheel_Trq_x=MDL.VehicleDynamics.SuspensionCompliance.Rear.Map_Angle_AlphaCamber_Wheel_Trq_x_2d  Map_Angle_Alpha_Wheel_Trq_y=MDL.VehicleDynamics.SuspensionCompliance.Rear.Map_Angle_AlphaCamber_Wheel_Trq_y_2d  Map_Angle_Alpha_Wheel_Trq_z=MDL.VehicleDynamics.SuspensionCompliance.Rear.Map_Angle_AlphaCamber_Wheel_Trq_z_2d  Map_Angle_Gamma_Wheel_F_x=MDL.VehicleDynamics.SuspensionCompliance.Rear.Map_Angle_GammaToe_Wheel_F_x_2d  Map_Angle_Gamma_Wheel_F_y=MDL.VehicleDynamics.SuspensionCompliance.Rear.Map_Angle_GammaToe_Wheel_F_y_2d  Map_Angle_Gamma_Wheel_Trq_x=MDL.VehicleDynamics.SuspensionCompliance.Rear.Map_Angle_GammaToe_Wheel_Trq_x_2d  Map_Angle_Gamma_Wheel_Trq_y=MDL.VehicleDynamics.SuspensionCompliance.Rear.Map_Angle_GammaToe_Wheel_Trq_y_2d  Map_Angle_Gamma_Wheel_Trq_z=MDL.VehicleDynamics.SuspensionCompliance.Rear.Map_Angle_GammaToe_Wheel_Trq_z_2d  Const_NaturalFrequency_Displ_x=MDL.VehicleDynamics.SuspensionCompliance.Rear.Const_NaturalFrequency_Displ_x  Const_NaturalFrequency_Displ_y=MDL.VehicleDynamics.SuspensionCompliance.Rear.Const_NaturalFrequency_Displ_y  Const_NaturalFrequency_Angle_Alpha=MDL.VehicleDynamics.SuspensionCompliance.Rear.Const_NaturalFrequency_Angle_AlphaCamber  Const_NaturalFrequency_Angle_Gamma=MDL.VehicleDynamics.SuspensionCompliance.Rear.Const_NaturalFrequency_Angle_GammaToe  StepSize=SIM.StepSize  ASMProperties=struct('Name','SUSCOMP_2D_REAR','Version','4.0','Library','ASM_VehicleDynamics_lib')  ASMInstanceName=suscomp_2d_rear  ASMInstanceID=1
  SUSPENSION_FORCES_REAR : ASM_VehicleDynamics_lib/VehicleDynamics/Suspension/Rear/CommonSuspensionBlocks/SUSPENSION_FORCES_REAR  Tag=ASM_SUBCOMPONENT  Map_Force_Left_Spring=MDL.VehicleDynamics.Suspension.Rear.Map_Force_LeftSpring  Map_Force_Left_Damper=MDL.VehicleDynamics.Suspension.Rear.Map_Force_LeftDamper  Map_Force_Right_Spring=MDL.VehicleDynamics.Suspension.Rear.Map_Force_RightSpring  Map_Force_Right_Damper=MDL.VehicleDynamics.Suspension.Rear.Map_Force_RightDamper  Map_Force_Stabilizer=MDL.VehicleDynamics.Suspension.Rear.Map_Force_Stabilizer  ASMProperties=struct('Name','SUSPENSION_FORCES_REAR','Version','4.0','Library','ASM_VehicleDynamics_lib')  ASMInstanceName=SusForcesRear  ASMInstanceID=1
  SUSPENSION_FORCE_KINEMATICS_REAR : ASM_VehicleDynamics_lib/VehicleDynamics/Suspension/Rear/CommonSuspensionBlocks/SUSPENSION_FORCE_KINEMATICS_REAR  Tag=ASM_SUBCOMPONENT  StepSize=SIM.StepSize  ASMProperties=struct('Name','SUSPENSION_FORCE_KINEMATICS_REAR','Version','5.0','Library','ASM_VehicleDynamics_lib')  ASMInstanceName=suspension_force_kinematics_rear  ASMInstanceID=1
  Selector1 : Selector  InputPortWidth=12  IndexOptions=Index vector (dialog)  Indices=[8 11]  OutputSizes=1
  Selector11 : Selector  InputPortWidth=12  IndexOptions=Index vector (dialog)  Indices=[7 10]  OutputSizes=1
  Selector4 : Selector  InputPortWidth=4  IndexOptions=Index vector (dialog)  Indices=[3 4]  OutputSizes=1
  Selector5 : Selector  InputPortWidth=12  IndexOptions=Index vector (dialog)  Indices=[7 10]  OutputSizes=1
  Selector6 : Selector  InputPortWidth=12  IndexOptions=Index vector (dialog)  Indices=[8 11]  OutputSizes=1
  Selector7 : Selector  InputPortWidth=12  IndexOptions=Index vector (dialog)  Indices=[9 12]  OutputSizes=1
  Selector9 : Selector  InputPortWidth=4  IndexOptions=Index vector (dialog)  Indices=[3 4]  OutputSizes=1
  Sum{,1..3} (4 alike) : Sum  Inputs=++|
  SusKin_Rear : Subsystem  Tag=VehicleDynamics_Suspension
  Terminator{,1..3} (4 alike) : Terminator
  WheelPos_Offset[x;y;z][m] : Constant  Value=[0 0 0]
  zeros : Constant  Value=zeros(6,1)
  "Pos_Wheel[RL;RR][x;y;z][m] " : Outport  VectorParamsAs1DForOutWhenUnconnected=off
  UnitVec_y_Wheel_CoorSys_V[RL;RR][x;y;z][] : Outport  Port=2  VectorParamsAs1DForOutWhenUnconnected=off
  v_Rel_WheelBody[RL;RR][x;y;z][m|s] : Outport  Port=3  VectorParamsAs1DForOutWhenUnconnected=off
  w_Rel_WheelBody[RL,RR][x;y;z][rad|s] : Outport  Port=4  VectorParamsAs1DForOutWhenUnconnected=off
  gF_Rear_Susp[q1,q2][] : Outport  Port=5  VectorParamsAs1DForOutWhenUnconnected=off
  gRear_dq_Rear_dt[2x2][] : Outport  Port=6  VectorParamsAs1DForOutWhenUnconnected=off
  SuspensionKinematicRelations_Rear : Outport  Port=7  VectorParamsAs1DForOutWhenUnconnected=off
  AirSuspensionSignals_Rear : Outport  Port=8  VectorParamsAs1DForOutWhenUnconnected=off
  ASMSignalBus : Outport  Port=9  VectorParamsAs1DForOutWhenUnconnected=off
  tag scope: ASMBUS_SuspensionComplianceRear=scoped, ASMBUS_SuspensionForceKinematicsRear=scoped, ASMBUS_SuspensionForcesRear=scoped, ASMBUS_SuspensionKinematicsRear=scoped, ASMBUS_SuspensionRelativePositionRear=scoped, ASMBUS_SuspensionRelativeVelocitiesRear=scoped
  wires:
  SusKin_Rear/24(Displ_Stabilizer_dSteering[Left;Right][]) -> Terminator3/1
  SusKin_Rear/23(Displ_Damper_dSteering[Left;Right][]) -> Terminator2/1
  SusKin_Rear/22(Displ_Spring_dSteering[Left;Right][]) -> Terminator1/1
  Selector4/1 -> SusKin_Rear/3(Displ_z_Wheel[Left;Right][m])
  SUSCOMP_2D_REAR/1 -> [ASMBUS_SuspensionComplianceRear]
  Constant/1 -> SusKin_Rear/2(Displ_SteeringRod_dt[Left;Right][m|s]), SusKin_Rear/1(Displ_SteeringRod[Left;Right][m]), RELATIVE_VELOCITIES_REAR/1
  RELATIVE_VELOCITIES_REAR/1 -> [ASMBUS_SuspensionRelativeVelocitiesRear]
  SUSCOMP_2D_REAR/2 -> RELATIVE_VELOCITIES_REAR/4
  SUSCOMP_2D_REAR/3 -> RELATIVE_VELOCITIES_REAR/5
  SUSCOMP_2D_REAR/4 -> RELATIVE_VELOCITIES_REAR/6
  SUSCOMP_2D_REAR/5 -> RELATIVE_VELOCITIES_REAR/7
  SUSCOMP_2D_REAR/6 -> RELATIVE_POSITION_REAR/1
  SUSCOMP_2D_REAR/7 -> RELATIVE_POSITION_REAR/2
  SUSCOMP_2D_REAR/8 -> RELATIVE_POSITION_REAR/3
  SUSCOMP_2D_REAR/9 -> RELATIVE_POSITION_REAR/4
  SusKin_Rear/10(Pos_Left_Wheel[x;y;z][m]) -> RELATIVE_POSITION_REAR/5
  SusKin_Rear/11(Pos_Right_Wheel[x;y;z][m]) -> RELATIVE_POSITION_REAR/6
  SusKin_Rear/12(UnitVec_y_Wheel_Left[x;y;z]) -> RELATIVE_POSITION_REAR/7
  SusKin_Rear/13(UnitVec_y_Wheel_Right[x;y;z]) -> RELATIVE_POSITION_REAR/8
  SusKin_Rear/14(Displ_Spring[Left;Right][m]) -> SUSPENSION_FORCES_REAR/1
  SusKin_Rear/15(Displ_Damper_dt[Left;Right][m|s]) -> SUSPENSION_FORCES_REAR/2
  SusKin_Rear/16(Displ_Stabilizer[m]) -> SUSPENSION_FORCES_REAR/3
  SUSPENSION_FORCES_REAR/4 -> SUSPENSION_FORCE_KINEMATICS_REAR/3
  SUSPENSION_FORCES_REAR/5 -> SUSPENSION_FORCE_KINEMATICS_REAR/4
  SUSPENSION_FORCES_REAR/6 -> SUSPENSION_FORCE_KINEMATICS_REAR/5
  SUSPENSION_FORCES_REAR/7 -> SUSPENSION_FORCE_KINEMATICS_REAR/6
  SUSPENSION_FORCES_REAR/10 -> SUSPENSION_FORCE_KINEMATICS_REAR/9
  SUSPENSION_FORCES_REAR/11 -> SUSPENSION_FORCE_KINEMATICS_REAR/10
  SusKin_Rear/17(Displ_Spring_Left_dq[qL;qR][]) -> SUSPENSION_FORCE_KINEMATICS_REAR/11
  SusKin_Rear/18(Displ_Damper_Left_dq[qL;qR][]) -> SUSPENSION_FORCE_KINEMATICS_REAR/12
  SusKin_Rear/19(Displ_Stabilizer_dq[qL;qR][]) -> SUSPENSION_FORCE_KINEMATICS_REAR/13
  SusKin_Rear/20(Displ_Spring_Right_dq[qL;qR][]) -> SUSPENSION_FORCE_KINEMATICS_REAR/14
  SusKin_Rear/21(Displ_Damper_Right_dq[qL;qR][]) -> SUSPENSION_FORCE_KINEMATICS_REAR/15
  SUSPENSION_FORCE_KINEMATICS_REAR/2 -> Mux1/1
  SUSPENSION_FORCE_KINEMATICS_REAR/3 -> Mux1/2
  Mux1/1 -> gF_Rear_Susp[q1,q2][]/1
  SUSPENSION_FORCE_KINEMATICS_REAR/4 -> gRear_dq_Rear_dt[2x2][]/1
  q_Wheel_dt[q1_Front;q2_Front;q1_Rear;q2_Rear][]/1 -> Selector9/1
  q_Wheel[q1_Front;q2_Front;q1_Rear;q2_Rear][]/1 -> Selector4/1
  SusKin_Rear/2(Pos_Left_Wheel_dq[qL;qR][x;y;z][]) -> Bus Creator/1, RELATIVE_VELOCITIES_REAR/8  "Pos_RL_Wheel_dq_Rear[q1;q2][x;y;z][]"
  SusKin_Rear/3(Pos_Left_Wheel_dDispl_SteeringRod[x;y;z][]) -> Bus Creator/2, RELATIVE_VELOCITIES_REAR/9  "Pos_RL_Wheel_dDispl_SteeringRod[x;y;z][]"
  SusKin_Rear/4(w_Rel_Left_Wheel_dq_dt[qL;qR][x;y;z][rad|m]) -> Bus Creator/3, RELATIVE_VELOCITIES_REAR/10  "w_Rel_RL_Wheel_dq_Rear_dt[q1;q2][x;y;z][]"
  SusKin_Rear/5(w_Rel_Left_Wheel_dDispl_SteeringRod_dt[x;y;z][rad|m]) -> Bus Creator/4, RELATIVE_VELOCITIES_REAR/11  "w_Rel_RL_Wheel_dDispl_SteeringRod_dt[x;y;z][rad|m]"
  SusKin_Rear/6(Pos_Right_Wheel_dq[qL;qR][x;y;z][]) -> Bus Creator/5, RELATIVE_VELOCITIES_REAR/12  "Pos_RR_Wheel_dq_Rear[q1;q2][x;y;z][]"
  SusKin_Rear/7(Pos_Right_Wheel_dDispl_SteeringRod[x;y;z][]) -> Bus Creator/6, RELATIVE_VELOCITIES_REAR/13  "Pos_RR_Wheel_dDispl_SteeringRod[x;y;z][]"
  SusKin_Rear/8(w_Rel_Right_Wheel_dq_dt[qL;qR][x;y;z][rad|m]) -> Bus Creator/7, RELATIVE_VELOCITIES_REAR/14  "w_Rel_RR_Wheel_dq_Rear[q1;q2][x;y;z][]"
  SusKin_Rear/9(w_Rel_Right_Wheel_dDispl_SteeringRod_dt[x;y;z][rad|m]) -> Bus Creator/8, RELATIVE_VELOCITIES_REAR/15  "w_Rel_RR_Wheel_dDispl_SteeringRod_dt[x;y;z][rad|m]"
  Bus Creator/1 -> SuspensionKinematicRelations_Rear/1  "SuspensionKinematicRelations_Rear"
  F_Tire[FL;FR;RL;RR][x;y;z][N]/1 -> Selector5/1, Selector6/1
  SUSPENSION_FORCES_REAR/1 -> [ASMBUS_SuspensionForcesRear]
  SUSPENSION_FORCE_KINEMATICS_REAR/1 -> [ASMBUS_SuspensionForceKinematicsRear]
  RELATIVE_POSITION_REAR/2 -> "Pos_Wheel[RL;RR][x;y;z][m] "/1
  RELATIVE_POSITION_REAR/3 -> UnitVec_y_Wheel_CoorSys_V[RL;RR][x;y;z][]/1
  RELATIVE_VELOCITIES_REAR/2 -> v_Rel_WheelBody[RL;RR][x;y;z][m|s]/1
  RELATIVE_VELOCITIES_REAR/3 -> w_Rel_WheelBody[RL,RR][x;y;z][rad|s]/1
  RELATIVE_POSITION_REAR/1 -> [ASMBUS_SuspensionRelativePositionRear]
  Demux/1 -> RELATIVE_VELOCITIES_REAR/2
  Demux/2 -> RELATIVE_VELOCITIES_REAR/3
  SusKin_Rear/1(ASMSignalBus) -> [ASMBUS_SuspensionKinematicsRear]
  WheelPos_Offset[x;y;z][m]/1 -> SusKin_Rear/5(WheelPos_Offset[x;y;z][m])
  Reset[]/1 -> SUSCOMP_2D_REAR/6
  Trq_Tire[FL;FR;RL;RR][x;y;z][Nm]/1 -> Selector11/1, Selector7/1, Selector1/1
  Constant2/1 -> SUSPENSION_FORCE_KINEMATICS_REAR/18, SUSPENSION_FORCE_KINEMATICS_REAR/19, SUSPENSION_FORCE_KINEMATICS_REAR/17, SUSPENSION_FORCE_KINEMATICS_REAR/16
  Constant3/1 -> SUSPENSION_FORCE_KINEMATICS_REAR/20, SUSPENSION_FORCE_KINEMATICS_REAR/21
  Sw_Rotation[1Cardan|2ToeCamberCaster]/1 -> RELATIVE_POSITION_REAR/9, SusKin_Rear/6(Sw_Rotation[1Cardan|2ToeCamberSideView]), SUSCOMP_2D_REAR/7
  zeros/1 -> SUSCOMP_2D_REAR/8
  Selector9/1 -> SusKin_Rear/4(Displ_z_dt_Wheel[Left;Right][m|s]), Demux/1
  Selector5/1 -> SUSCOMP_2D_REAR/1
  Selector6/1 -> SUSCOMP_2D_REAR/2
  Selector11/1 -> SUSCOMP_2D_REAR/3
  Selector7/1 -> SUSCOMP_2D_REAR/5
  SUSPENSION_FORCES_REAR/2 -> Sum/2
  SUSPENSION_FORCES_REAR/3 -> Sum1/2
  SUSPENSION_FORCES_REAR/8 -> Sum2/2
  SUSPENSION_FORCES_REAR/9 -> Sum3/2
  Sum/1 -> SUSPENSION_FORCE_KINEMATICS_REAR/1
  F_RL_external[N]/1 -> Sum/1
  Sum1/1 -> SUSPENSION_FORCE_KINEMATICS_REAR/2
  F_RL_dDispl_external[N|m]/1 -> Sum1/1
  F_RR_external[N]/1 -> Sum2/1
  F_RR_dDispl_external[N|m]/1 -> Sum3/1
  Sum2/1 -> SUSPENSION_FORCE_KINEMATICS_REAR/7
  Sum3/1 -> SUSPENSION_FORCE_KINEMATICS_REAR/8
  AirSuspensionSignals_In/1 -> Terminator/1
  Constant1/1 -> AirSuspensionSignals_Rear/1
  Selector1/1 -> SUSCOMP_2D_REAR/4
  ASMSignalCollector/1(SuspensionRear) -> ASMSignalBus/1
